simulink model "scheme_L2"  (R2025b)
settings: Solver=VariableStepAuto  StartTime=0.0  StopTime=20  MaxStep=0.02  RelTol=1e-3
settings Model: Creator=Sonya  LastModifiedBy=Sonya

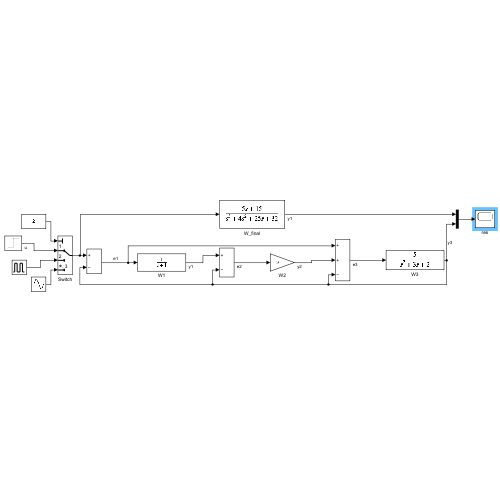
[thumbnail: Simulink's stored preview of the top-level diagram]
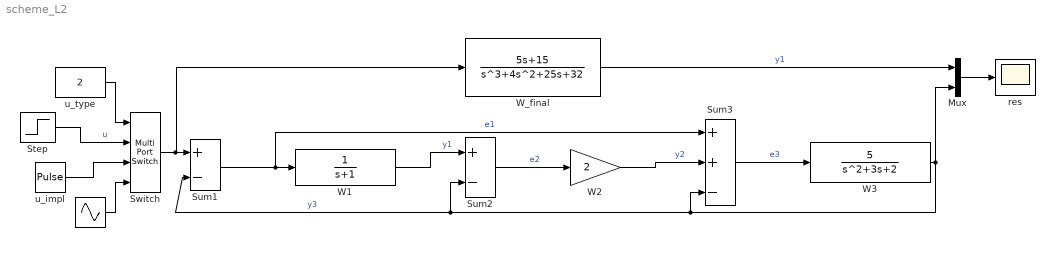
== system scheme_L2 ==
  " " : Sin  Frequency=3  SampleTime=0
  Mux : Mux  Inputs=2
  Step : Step  SampleTime=0
  Sum1 : Sum  Inputs=+-
  Sum2 : Sum  Inputs=+-
  Sum3 : Sum  Inputs=++-
  Switch : MultiPortSwitch
  W1 : TransferFcn  Numerator=1  Denominator=[1 1]
  W2 : Gain  Gain=2
  W3 : TransferFcn  Numerator=5  Denominator=[1 3 2]
  W_final : TransferFcn  Numerator=[5 15]  Denominator=[1 4 25 32]
  res : Scope
      settings: ActiveDisplayYMinimum=-0.30397842960699079  ActiveDisplayYMaximum=0.88761922626807133
  u_impl : DiscretePulseGenerator  PulseType=Time based  Amplitude=20  Period=20  PulseWidth=0.2  PhaseDelay=2
  u_type : Constant  Value=2
  wires:
  Sum1/1 -> W1/1, Sum3/1  "e1"
  W1/1 -> Sum2/1  "y1"
  Sum2/1 -> W2/1  "e2"
  W2/1 -> Sum3/2  "y2"
  Sum3/1 -> W3/1  "e3"
  W3/1 -> Mux/2, Sum1/2, Sum2/2, Sum3/3  "y3"
  Mux/1 -> res/1
  W_final/1 -> Mux/1  "y1"
  Switch/1 -> W_final/1, Sum1/1
  u_type/1 -> Switch/1
  Step/1 -> Switch/2  "u"
  u_impl/1 -> Switch/3
  " "/1 -> Switch/4
